simulink model "fft_biplex_real_4x_delay_bram_test"  (Simulink 7.4)
settings: Solver=VariableStepDiscrete  StartTime=0.0  StopTime=256  RelTol=1e-3
libraries: xbsIndex_r4 x596, casper_library_misc x36, casper_library_delays x8, casper_library_ffts_twiddle x1, simulink x1
(part 6 of 6)

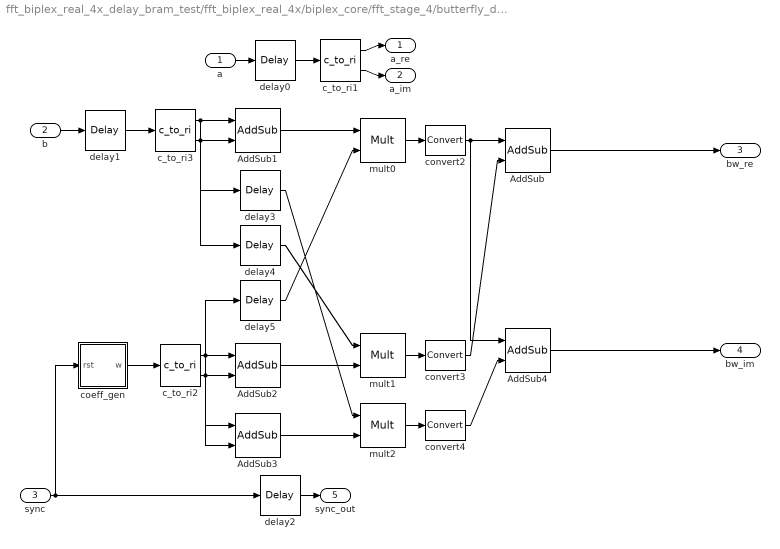
== system fft_biplex_real_4x_delay_bram_test/fft_biplex_real_4x/biplex_core/fft_stage_4/butterfly_direct/twiddle_general_3mult ==
  a : Inport
  b : Inport  Port=2
  sync : Inport  Port=3
  AddSub : xbsIndex_r4/AddSub  mode=Subtraction  use_carryin=off  use_carryout=off  en=off  latency=add_latency  precision=Full  arith_type=Unsigned  n_bits=16  bin_pt=14  quantization=Truncate  overflow=Wrap  dbl_ovrd=off  use_behavioral_HDL=on  hw_selection=Fabric  pipelined=off  block_type=addsub
  AddSub1 : xbsIndex_r4/AddSub  mode=Addition  use_carryin=off  use_carryout=off  en=off  latency=add_latency  precision=Full  arith_type=Unsigned  n_bits=16  bin_pt=14  quantization=Truncate  overflow=Wrap  dbl_ovrd=off  use_behavioral_HDL=on  hw_selection=Fabric  pipelined=off  block_type=addsub
  AddSub2 : xbsIndex_r4/AddSub  mode=Addition  use_carryin=off  use_carryout=off  en=off  latency=add_latency  precision=Full  arith_type=Unsigned  n_bits=16  bin_pt=14  quantization=Truncate  overflow=Wrap  dbl_ovrd=off  use_behavioral_HDL=on  hw_selection=Fabric  pipelined=off  block_type=addsub
  AddSub3 : xbsIndex_r4/AddSub  mode=Subtraction  use_carryin=off  use_carryout=off  en=off  latency=add_latency  precision=Full  arith_type=Unsigned  n_bits=16  bin_pt=14  quantization=Truncate  overflow=Wrap  dbl_ovrd=off  use_behavioral_HDL=on  hw_selection=Fabric  pipelined=off  block_type=addsub
  AddSub4 : xbsIndex_r4/AddSub  mode=Addition  use_carryin=off  use_carryout=off  en=off  latency=add_latency  precision=Full  arith_type=Unsigned  n_bits=16  bin_pt=14  quantization=Truncate  overflow=Wrap  dbl_ovrd=off  use_behavioral_HDL=on  hw_selection=Fabric  pipelined=off  block_type=addsub
  c_to_ri1 : casper_library_misc/c_to_ri  SystemSampleTime=-1  n_bits=16  bin_pt=15
      settings: AttributesFormatString=16_15 r/i
  c_to_ri2 : casper_library_misc/c_to_ri  SystemSampleTime=-1  n_bits=15  bin_pt=13
      settings: AttributesFormatString=15_13 r/i
  c_to_ri3 : casper_library_misc/c_to_ri  SystemSampleTime=-1  n_bits=input_bit_width  bin_pt=input_bit_width-1
      settings: AttributesFormatString=16_15 r/i
  coeff_gen : Subsystem  AncestorBlock=casper_library_ffts_twiddle_coeff_gen/coeff_gen  mask(coeff_gen){Coeffs=[1+0i                                        6.123233995736766035868820147292e-17-1i         0.70710678118654757273731092936941-0.70710678118654746171500846685376i        -0.70710678118654746171500846685376-0.70710678118654757273731092936941i         0.92387953251128673848313610506011-0.38268343236508978177923268049199i        -0.38268343236508972626808144923416-0.92387953251128673848313610506011i         0.38268343236508983729038391174981-0.92387953251128673848313610506011i        -0.92387953251128673848313610506011-0.38268343236508989280153514300764i], coeff_bit_width=15, StepPeriod=1, bram_latency=bram_latency, coeffs_bram=off}
      mask prompts: Coeffs "Coefficients: (0 to 2^(FFTSize-1)-1)"; coeff_bit_width "Coefficient Bit Width:"; StepPeriod "Step Period: (2^?)"; bram_latency "Latency:"; coeffs_bram "Store coefficients in BRAM"
      mask help: Generates a sequence of complex coefficients
      mask init:
      | coeff_gen_init( gcb, ...
      |     'Coeffs', Coeffs, ...
      |     'coeff_bit_width', coeff_bit_width, ...
      |     'StepPeriod', StepPeriod, ...
      |     'bram_latency', bram_latency, ...
      |     'coeffs_bram', coeffs_bram);
      settings: AttributesFormatString=8 @ (15,13)
      mask CallbackString:
      | Coeffs = eval(get_param(gcb, 'Coeffs'));
      | if( length(Coeffs) == 1 ),
      |     set_param(gcb, 'MaskVisibilities',{'on','on','off','off','off'});
      | else
      |     set_param(gcb, 'MaskVisibilities',{'on','on','on','on','on'});
      | end||||
  convert2 : xbsIndex_r4/Convert  arith_type="Signed  (2's comp)"  n_bits=input_bit_width+4  bin_pt=input_bit_width+1  quantization=Truncate  overflow=Saturate  latency=conv_latency  dbl_ovrd=off  pipeline=on  block_type=convert
      settings: block_version=11.4
  convert3 : xbsIndex_r4/Convert  arith_type="Signed  (2's comp)"  n_bits=input_bit_width+4  bin_pt=input_bit_width+1  quantization=Truncate  overflow=Saturate  latency=conv_latency  dbl_ovrd=off  pipeline=on  block_type=convert
      settings: block_version=11.4
  convert4 : xbsIndex_r4/Convert  arith_type="Signed  (2's comp)"  n_bits=input_bit_width+4  bin_pt=input_bit_width+1  quantization=Truncate  overflow=Saturate  latency=conv_latency  dbl_ovrd=off  pipeline=on  block_type=convert
      settings: block_version=11.4
  delay0 : xbsIndex_r4/Delay  en=off  latency=mult_latency + 2*add_latency + bram_latency + conv_latency  dbl_ovrd=off  reg_retiming=off  block_type=delay
      settings: block_version=11.4
  delay1 : xbsIndex_r4/Delay  en=off  latency=bram_latency  dbl_ovrd=off  reg_retiming=off  block_type=delay
      settings: block_version=11.4
  delay2 : xbsIndex_r4/Delay  en=off  latency=mult_latency + 2*add_latency + bram_latency + conv_latency  dbl_ovrd=off  reg_retiming=off  block_type=delay
      settings: block_version=11.4
  delay3 : xbsIndex_r4/Delay  en=off  latency=add_latency  dbl_ovrd=off  reg_retiming=on  block_type=delay
      settings: block_version=11.4
  delay4 : xbsIndex_r4/Delay  en=off  latency=add_latency  dbl_ovrd=off  reg_retiming=on  block_type=delay
      settings: block_version=11.4
  delay5 : xbsIndex_r4/Delay  en=off  latency=add_latency  dbl_ovrd=off  reg_retiming=on  block_type=delay
      settings: block_version=11.4
  mult0 : xbsIndex_r4/Mult  precision=Full  arith_type="Signed  (2's comp)"  n_bits=16  bin_pt=14  quantization=Truncate  overflow=Wrap  en=off  latency=mult_latency  dbl_ovrd=off  use_behavioral_HDL=on  opt=Speed  use_embedded=off  optimum_pipeline=off  pipeline=on  use_rpm=on  placement_style=Triangular  block_type=mult
      settings: block_version=11.4
  mult1 : xbsIndex_r4/Mult  precision=Full  arith_type="Signed  (2's comp)"  n_bits=16  bin_pt=14  quantization=Truncate  overflow=Wrap  en=off  latency=mult_latency  dbl_ovrd=off  use_behavioral_HDL=on  opt=Speed  use_embedded=off  optimum_pipeline=off  pipeline=on  use_rpm=on  placement_style=Triangular  block_type=mult
      settings: block_version=11.4
  mult2 : xbsIndex_r4/Mult  precision=Full  arith_type="Signed  (2's comp)"  n_bits=16  bin_pt=14  quantization=Truncate  overflow=Wrap  en=off  latency=mult_latency  dbl_ovrd=off  use_behavioral_HDL=on  opt=Speed  use_embedded=off  optimum_pipeline=off  pipeline=on  use_rpm=on  placement_style=Triangular  block_type=mult
      settings: block_version=11.4
  a_re : Outport
  a_im : Outport  Port=2
  bw_re : Outport  Port=3
  bw_im : Outport  Port=4
  sync_out : Outport  Port=5
  wires:
  a/1 -> delay0/1
  delay0/1 -> c_to_ri1/1
  c_to_ri1/1 -> a_re/1
  c_to_ri1/2 -> a_im/1
  sync/1 -> delay2/1, coeff_gen/1(rst)
  delay2/1 -> sync_out/1
  coeff_gen/1(w) -> c_to_ri2/1
  c_to_ri2/1 -> AddSub2/1, AddSub3/2, delay5/1
  c_to_ri2/2 -> AddSub2/2, AddSub3/1
  b/1 -> delay1/1
  delay1/1 -> c_to_ri3/1
  c_to_ri3/1 -> AddSub1/1, delay3/1
  c_to_ri3/2 -> AddSub1/2, delay4/1
  AddSub1/1 -> mult0/1
  delay5/1 -> mult0/2
  delay4/1 -> mult1/1
  AddSub2/1 -> mult1/2
  delay3/1 -> mult2/1
  AddSub3/1 -> mult2/2
  mult0/1 -> convert2/1
  mult1/1 -> convert3/1
  mult2/1 -> convert4/1
  convert2/1 -> AddSub/1, AddSub4/1
  convert3/1 -> AddSub/2
  convert4/1 -> AddSub4/2
  AddSub/1 -> bw_re/1
  AddSub4/1 -> bw_im/1

== system fft_biplex_real_4x_delay_bram_test/fft_biplex_real_4x/biplex_core/fft_stage_5/butterfly_direct/convert_of0 ==
  din : Inport  OutDataType=sfix(16)  OutScaling=2^0
  all_0s : xbsIndex_r4/Logical  logical_function=NAND  inputs=5  en=off  latency=latency  precision=Full  arith_type=Unsigned  n_bits=16  bin_pt=0  align_bp=on  dbl_ovrd=off  block_type=logical
  all_1s : xbsIndex_r4/Logical  logical_function=NAND  inputs=5  en=off  latency=latency  precision=Full  arith_type=Unsigned  n_bits=16  bin_pt=0  align_bp=on  dbl_ovrd=off  block_type=logical
  and : xbsIndex_r4/Logical  logical_function=AND  inputs=2  en=off  latency=0  precision=Full  arith_type=Unsigned  n_bits=16  bin_pt=0  align_bp=on  dbl_ovrd=off  block_type=logical
  convert : xbsIndex_r4/Convert  arith_type="Signed  (2's comp)"  n_bits=bit_width_o  bin_pt=binary_point_o  quantization=Truncate  overflow=Saturate  latency=latency  dbl_ovrd=off  pipeline=on  block_type=convert
      settings: block_version=10.1.1
  invert{1..5} (5 alike) : xbsIndex_r4/Inverter  en=off  latency=0  dbl_ovrd=off  block_type=inv
      invert3 settings: block_version=11.4
      invert4 settings: block_version=11.4
      invert5 settings: block_version=11.4
  slice1 : xbsIndex_r4/Slice  nbits=1  boolean_output=on  mode=Upper Bit Location + Width  bit1=0  base1=MSB of Input  bit0=0  base0=LSB of Input  dbl_ovrd=off  block_type=slice
      settings: infoedit="Extracts a given range of bits from each input sample and presents it at the output.  The output type is ordinarily unsigned with binary point at zero, but can be Boolean when the slice is one bit wide.<P><P>Hardware notes: In hardware this block costs nothing."  block_version=10.1.1
  slice2 : xbsIndex_r4/Slice  nbits=1  boolean_output=on  mode=Upper Bit Location + Width  bit1=-1  base1=MSB of Input  bit0=0  base0=LSB of Input  dbl_ovrd=off  block_type=slice
      settings: infoedit="Extracts a given range of bits from each input sample and presents it at the output.  The output type is ordinarily unsigned with binary point at zero, but can be Boolean when the slice is one bit wide.<P><P>Hardware notes: In hardware this block costs nothing."  block_version=10.1.1
  slice3 : xbsIndex_r4/Slice  nbits=1  boolean_output=on  mode=Upper Bit Location + Width  bit1=-2  base1=MSB of Input  bit0=0  base0=LSB of Input  dbl_ovrd=off  block_type=slice
  slice4 : xbsIndex_r4/Slice  nbits=1  boolean_output=on  mode=Upper Bit Location + Width  bit1=-3  base1=MSB of Input  bit0=0  base0=LSB of Input  dbl_ovrd=off  block_type=slice
  slice5 : xbsIndex_r4/Slice  nbits=1  boolean_output=on  mode=Upper Bit Location + Width  bit1=-4  base1=MSB of Input  bit0=0  base0=LSB of Input  dbl_ovrd=off  block_type=slice
  dout : Outport
  of : Outport  Port=2
  wires:
  din/1 -> convert/1, slice1/1, slice2/1, slice3/1, slice4/1, slice5/1
  convert/1 -> dout/1
  slice1/1 -> all_1s/1, invert1/1
  invert1/1 -> all_0s/1
  slice2/1 -> all_1s/2, invert2/1
  invert2/1 -> all_0s/2
  slice3/1 -> all_1s/3, invert3/1
  invert3/1 -> all_0s/3
  slice4/1 -> all_1s/4, invert4/1
  invert4/1 -> all_0s/4
  slice5/1 -> all_1s/5, invert5/1
  invert5/1 -> all_0s/5
  all_0s/1 -> and/1
  all_1s/1 -> and/2
  and/1 -> of/1

== system fft_biplex_real_4x_delay_bram_test/fft_biplex_real_4x/biplex_core/fft_stage_5/butterfly_direct/convert_of1 ==
  din : Inport  OutDataType=sfix(16)  OutScaling=2^0
  all_0s : xbsIndex_r4/Logical  logical_function=NAND  inputs=5  en=off  latency=latency  precision=Full  arith_type=Unsigned  n_bits=16  bin_pt=0  align_bp=on  dbl_ovrd=off  block_type=logical
  all_1s : xbsIndex_r4/Logical  logical_function=NAND  inputs=5  en=off  latency=latency  precision=Full  arith_type=Unsigned  n_bits=16  bin_pt=0  align_bp=on  dbl_ovrd=off  block_type=logical
  and : xbsIndex_r4/Logical  logical_function=AND  inputs=2  en=off  latency=0  precision=Full  arith_type=Unsigned  n_bits=16  bin_pt=0  align_bp=on  dbl_ovrd=off  block_type=logical
  convert : xbsIndex_r4/Convert  arith_type="Signed  (2's comp)"  n_bits=bit_width_o  bin_pt=binary_point_o  quantization=Truncate  overflow=Saturate  latency=latency  dbl_ovrd=off  pipeline=on  block_type=convert
      settings: block_version=10.1.1
  invert{1..5} (5 alike) : xbsIndex_r4/Inverter  en=off  latency=0  dbl_ovrd=off  block_type=inv
      invert3 settings: block_version=11.4
      invert4 settings: block_version=11.4
      invert5 settings: block_version=11.4
  slice1 : xbsIndex_r4/Slice  nbits=1  boolean_output=on  mode=Upper Bit Location + Width  bit1=0  base1=MSB of Input  bit0=0  base0=LSB of Input  dbl_ovrd=off  block_type=slice
      settings: infoedit="Extracts a given range of bits from each input sample and presents it at the output.  The output type is ordinarily unsigned with binary point at zero, but can be Boolean when the slice is one bit wide.<P><P>Hardware notes: In hardware this block costs nothing."  block_version=10.1.1
  slice2 : xbsIndex_r4/Slice  nbits=1  boolean_output=on  mode=Upper Bit Location + Width  bit1=-1  base1=MSB of Input  bit0=0  base0=LSB of Input  dbl_ovrd=off  block_type=slice
      settings: infoedit="Extracts a given range of bits from each input sample and presents it at the output.  The output type is ordinarily unsigned with binary point at zero, but can be Boolean when the slice is one bit wide.<P><P>Hardware notes: In hardware this block costs nothing."  block_version=10.1.1
  slice3 : xbsIndex_r4/Slice  nbits=1  boolean_output=on  mode=Upper Bit Location + Width  bit1=-2  base1=MSB of Input  bit0=0  base0=LSB of Input  dbl_ovrd=off  block_type=slice
  slice4 : xbsIndex_r4/Slice  nbits=1  boolean_output=on  mode=Upper Bit Location + Width  bit1=-3  base1=MSB of Input  bit0=0  base0=LSB of Input  dbl_ovrd=off  block_type=slice
  slice5 : xbsIndex_r4/Slice  nbits=1  boolean_output=on  mode=Upper Bit Location + Width  bit1=-4  base1=MSB of Input  bit0=0  base0=LSB of Input  dbl_ovrd=off  block_type=slice
  dout : Outport
  of : Outport  Port=2
  wires:
  din/1 -> convert/1, slice1/1, slice2/1, slice3/1, slice4/1, slice5/1
  convert/1 -> dout/1
  slice1/1 -> all_1s/1, invert1/1
  invert1/1 -> all_0s/1
  slice2/1 -> all_1s/2, invert2/1
  invert2/1 -> all_0s/2
  slice3/1 -> all_1s/3, invert3/1
  invert3/1 -> all_0s/3
  slice4/1 -> all_1s/4, invert4/1
  invert4/1 -> all_0s/4
  slice5/1 -> all_1s/5, invert5/1
  invert5/1 -> all_0s/5
  all_0s/1 -> and/1
  all_1s/1 -> and/2
  and/1 -> of/1

== system fft_biplex_real_4x_delay_bram_test/fft_biplex_real_4x/biplex_core/fft_stage_5/butterfly_direct/convert_of2 ==
  din : Inport  OutDataType=sfix(16)  OutScaling=2^0
  all_0s : xbsIndex_r4/Logical  logical_function=NAND  inputs=5  en=off  latency=latency  precision=Full  arith_type=Unsigned  n_bits=16  bin_pt=0  align_bp=on  dbl_ovrd=off  block_type=logical
  all_1s : xbsIndex_r4/Logical  logical_function=NAND  inputs=5  en=off  latency=latency  precision=Full  arith_type=Unsigned  n_bits=16  bin_pt=0  align_bp=on  dbl_ovrd=off  block_type=logical
  and : xbsIndex_r4/Logical  logical_function=AND  inputs=2  en=off  latency=0  precision=Full  arith_type=Unsigned  n_bits=16  bin_pt=0  align_bp=on  dbl_ovrd=off  block_type=logical
  convert : xbsIndex_r4/Convert  arith_type="Signed  (2's comp)"  n_bits=bit_width_o  bin_pt=binary_point_o  quantization=Truncate  overflow=Saturate  latency=latency  dbl_ovrd=off  pipeline=on  block_type=convert
      settings: block_version=10.1.1
  invert{1..5} (5 alike) : xbsIndex_r4/Inverter  en=off  latency=0  dbl_ovrd=off  block_type=inv
      invert3 settings: block_version=11.4
      invert4 settings: block_version=11.4
      invert5 settings: block_version=11.4
  slice1 : xbsIndex_r4/Slice  nbits=1  boolean_output=on  mode=Upper Bit Location + Width  bit1=0  base1=MSB of Input  bit0=0  base0=LSB of Input  dbl_ovrd=off  block_type=slice
      settings: infoedit="Extracts a given range of bits from each input sample and presents it at the output.  The output type is ordinarily unsigned with binary point at zero, but can be Boolean when the slice is one bit wide.<P><P>Hardware notes: In hardware this block costs nothing."  block_version=10.1.1
  slice2 : xbsIndex_r4/Slice  nbits=1  boolean_output=on  mode=Upper Bit Location + Width  bit1=-1  base1=MSB of Input  bit0=0  base0=LSB of Input  dbl_ovrd=off  block_type=slice
      settings: infoedit="Extracts a given range of bits from each input sample and presents it at the output.  The output type is ordinarily unsigned with binary point at zero, but can be Boolean when the slice is one bit wide.<P><P>Hardware notes: In hardware this block costs nothing."  block_version=10.1.1
  slice3 : xbsIndex_r4/Slice  nbits=1  boolean_output=on  mode=Upper Bit Location + Width  bit1=-2  base1=MSB of Input  bit0=0  base0=LSB of Input  dbl_ovrd=off  block_type=slice
  slice4 : xbsIndex_r4/Slice  nbits=1  boolean_output=on  mode=Upper Bit Location + Width  bit1=-3  base1=MSB of Input  bit0=0  base0=LSB of Input  dbl_ovrd=off  block_type=slice
  slice5 : xbsIndex_r4/Slice  nbits=1  boolean_output=on  mode=Upper Bit Location + Width  bit1=-4  base1=MSB of Input  bit0=0  base0=LSB of Input  dbl_ovrd=off  block_type=slice
  dout : Outport
  of : Outport  Port=2
  wires:
  din/1 -> convert/1, slice1/1, slice2/1, slice3/1, slice4/1, slice5/1
  convert/1 -> dout/1
  slice1/1 -> all_1s/1, invert1/1
  invert1/1 -> all_0s/1
  slice2/1 -> all_1s/2, invert2/1
  invert2/1 -> all_0s/2
  slice3/1 -> all_1s/3, invert3/1
  invert3/1 -> all_0s/3
  slice4/1 -> all_1s/4, invert4/1
  invert4/1 -> all_0s/4
  slice5/1 -> all_1s/5, invert5/1
  invert5/1 -> all_0s/5
  all_0s/1 -> and/1
  all_1s/1 -> and/2
  and/1 -> of/1

== system fft_biplex_real_4x_delay_bram_test/fft_biplex_real_4x/biplex_core/fft_stage_5/butterfly_direct/convert_of3 ==
  din : Inport  OutDataType=sfix(16)  OutScaling=2^0
  all_0s : xbsIndex_r4/Logical  logical_function=NAND  inputs=5  en=off  latency=latency  precision=Full  arith_type=Unsigned  n_bits=16  bin_pt=0  align_bp=on  dbl_ovrd=off  block_type=logical
  all_1s : xbsIndex_r4/Logical  logical_function=NAND  inputs=5  en=off  latency=latency  precision=Full  arith_type=Unsigned  n_bits=16  bin_pt=0  align_bp=on  dbl_ovrd=off  block_type=logical
  and : xbsIndex_r4/Logical  logical_function=AND  inputs=2  en=off  latency=0  precision=Full  arith_type=Unsigned  n_bits=16  bin_pt=0  align_bp=on  dbl_ovrd=off  block_type=logical
  convert : xbsIndex_r4/Convert  arith_type="Signed  (2's comp)"  n_bits=bit_width_o  bin_pt=binary_point_o  quantization=Truncate  overflow=Saturate  latency=latency  dbl_ovrd=off  pipeline=on  block_type=convert
      settings: block_version=10.1.1
  invert{1..5} (5 alike) : xbsIndex_r4/Inverter  en=off  latency=0  dbl_ovrd=off  block_type=inv
      invert3 settings: block_version=11.4
      invert4 settings: block_version=11.4
      invert5 settings: block_version=11.4
  slice1 : xbsIndex_r4/Slice  nbits=1  boolean_output=on  mode=Upper Bit Location + Width  bit1=0  base1=MSB of Input  bit0=0  base0=LSB of Input  dbl_ovrd=off  block_type=slice
      settings: infoedit="Extracts a given range of bits from each input sample and presents it at the output.  The output type is ordinarily unsigned with binary point at zero, but can be Boolean when the slice is one bit wide.<P><P>Hardware notes: In hardware this block costs nothing."  block_version=10.1.1
  slice2 : xbsIndex_r4/Slice  nbits=1  boolean_output=on  mode=Upper Bit Location + Width  bit1=-1  base1=MSB of Input  bit0=0  base0=LSB of Input  dbl_ovrd=off  block_type=slice
      settings: infoedit="Extracts a given range of bits from each input sample and presents it at the output.  The output type is ordinarily unsigned with binary point at zero, but can be Boolean when the slice is one bit wide.<P><P>Hardware notes: In hardware this block costs nothing."  block_version=10.1.1
  slice3 : xbsIndex_r4/Slice  nbits=1  boolean_output=on  mode=Upper Bit Location + Width  bit1=-2  base1=MSB of Input  bit0=0  base0=LSB of Input  dbl_ovrd=off  block_type=slice
  slice4 : xbsIndex_r4/Slice  nbits=1  boolean_output=on  mode=Upper Bit Location + Width  bit1=-3  base1=MSB of Input  bit0=0  base0=LSB of Input  dbl_ovrd=off  block_type=slice
  slice5 : xbsIndex_r4/Slice  nbits=1  boolean_output=on  mode=Upper Bit Location + Width  bit1=-4  base1=MSB of Input  bit0=0  base0=LSB of Input  dbl_ovrd=off  block_type=slice
  dout : Outport
  of : Outport  Port=2
  wires:
  din/1 -> convert/1, slice1/1, slice2/1, slice3/1, slice4/1, slice5/1
  convert/1 -> dout/1
  slice1/1 -> all_1s/1, invert1/1
  invert1/1 -> all_0s/1
  slice2/1 -> all_1s/2, invert2/1
  invert2/1 -> all_0s/2
  slice3/1 -> all_1s/3, invert3/1
  invert3/1 -> all_0s/3
  slice4/1 -> all_1s/4, invert4/1
  invert4/1 -> all_0s/4
  slice5/1 -> all_1s/5, invert5/1
  invert5/1 -> all_0s/5
  all_0s/1 -> and/1
  all_1s/1 -> and/2
  and/1 -> of/1

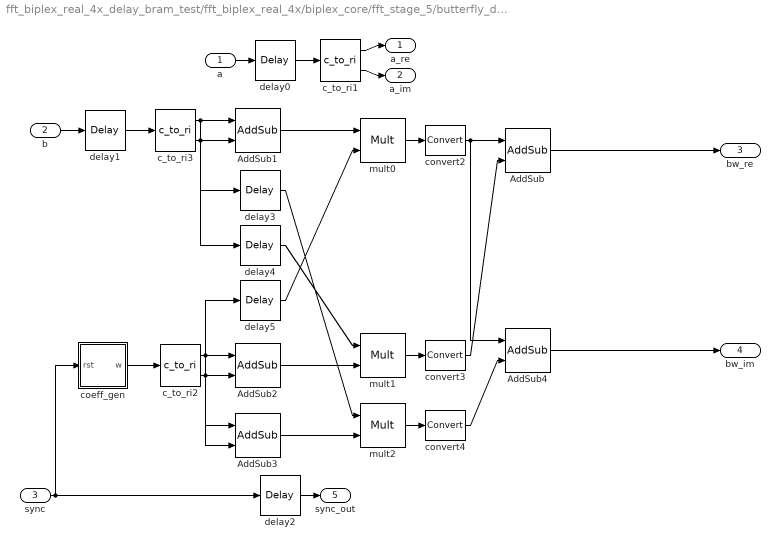
== system fft_biplex_real_4x_delay_bram_test/fft_biplex_real_4x/biplex_core/fft_stage_5/butterfly_direct/twiddle_general_3mult ==
  a : Inport
  b : Inport  Port=2
  sync : Inport  Port=3
  AddSub : xbsIndex_r4/AddSub  mode=Subtraction  use_carryin=off  use_carryout=off  en=off  latency=add_latency  precision=Full  arith_type=Unsigned  n_bits=16  bin_pt=14  quantization=Truncate  overflow=Wrap  dbl_ovrd=off  use_behavioral_HDL=on  hw_selection=Fabric  pipelined=off  block_type=addsub
  AddSub1 : xbsIndex_r4/AddSub  mode=Addition  use_carryin=off  use_carryout=off  en=off  latency=add_latency  precision=Full  arith_type=Unsigned  n_bits=16  bin_pt=14  quantization=Truncate  overflow=Wrap  dbl_ovrd=off  use_behavioral_HDL=on  hw_selection=Fabric  pipelined=off  block_type=addsub
  AddSub2 : xbsIndex_r4/AddSub  mode=Addition  use_carryin=off  use_carryout=off  en=off  latency=add_latency  precision=Full  arith_type=Unsigned  n_bits=16  bin_pt=14  quantization=Truncate  overflow=Wrap  dbl_ovrd=off  use_behavioral_HDL=on  hw_selection=Fabric  pipelined=off  block_type=addsub
  AddSub3 : xbsIndex_r4/AddSub  mode=Subtraction  use_carryin=off  use_carryout=off  en=off  latency=add_latency  precision=Full  arith_type=Unsigned  n_bits=16  bin_pt=14  quantization=Truncate  overflow=Wrap  dbl_ovrd=off  use_behavioral_HDL=on  hw_selection=Fabric  pipelined=off  block_type=addsub
  AddSub4 : xbsIndex_r4/AddSub  mode=Addition  use_carryin=off  use_carryout=off  en=off  latency=add_latency  precision=Full  arith_type=Unsigned  n_bits=16  bin_pt=14  quantization=Truncate  overflow=Wrap  dbl_ovrd=off  use_behavioral_HDL=on  hw_selection=Fabric  pipelined=off  block_type=addsub
  c_to_ri1 : casper_library_misc/c_to_ri  SystemSampleTime=-1  n_bits=16  bin_pt=15
      settings: AttributesFormatString=16_15 r/i
  c_to_ri2 : casper_library_misc/c_to_ri  SystemSampleTime=-1  n_bits=15  bin_pt=13
      settings: AttributesFormatString=15_13 r/i
  c_to_ri3 : casper_library_misc/c_to_ri  SystemSampleTime=-1  n_bits=input_bit_width  bin_pt=input_bit_width-1
      settings: AttributesFormatString=16_15 r/i
  coeff_gen : Subsystem  AncestorBlock=casper_library_ffts_twiddle_coeff_gen/coeff_gen  mask(coeff_gen){Coeffs=[1+0i                                        6.123233995736766035868820147292e-17-1i         0.70710678118654757273731092936941-0.70710678118654746171500846685376i        -0.70710678118654746171500846685376-0.70710678118654757273731092936941i         0.92387953251128673848313610506011-0.38268343236508978177923268049199i        -0.38268343236508972626808144923416-0.92387953251128673848313610506011i         0.38268343236508983729038391174981-0.92387953251128673848313610506011i        -0.92387953251128673848313610506011-0.38268343236508989280153514300764i         0.98078528040323043057924223830923-0.19509032201612824808378832130984i        -0.19509032201612819257263709005201-0.98078528040323043057924223830923i          0.55557023301960228867102387084742-0.8314696123025452356714026791451i        -0.83146961230254534669370514166076-0.55557023301960217764872140833177i          0.8314696123025452356714026791451-0.55557023301960217764872140833177i        -0.55557023301960195560411648330046-0.83146961230254534669370514166076i         0.19509032201612833135051516819658-0.98078528040323043057924223830923i        -0.98078528040323043057924223830923-0.19509032201612860890627132448572i], coeff_bit_width=15, StepPeriod=0, bram_latency=bram_latency, coeffs_bram=off}
      mask prompts: Coeffs "Coefficients: (0 to 2^(FFTSize-1)-1)"; coeff_bit_width "Coefficient Bit Width:"; StepPeriod "Step Period: (2^?)"; bram_latency "Latency:"; coeffs_bram "Store coefficients in BRAM"
      mask help: Generates a sequence of complex coefficients
      mask init:
      | coeff_gen_init( gcb, ...
      |     'Coeffs', Coeffs, ...
      |     'coeff_bit_width', coeff_bit_width, ...
      |     'StepPeriod', StepPeriod, ...
      |     'bram_latency', bram_latency, ...
      |     'coeffs_bram', coeffs_bram);
      settings: AttributesFormatString=16 @ (15,13)
      mask CallbackString:
      | Coeffs = eval(get_param(gcb, 'Coeffs'));
      | if( length(Coeffs) == 1 ),
      |     set_param(gcb, 'MaskVisibilities',{'on','on','off','off','off'});
      | else
      |     set_param(gcb, 'MaskVisibilities',{'on','on','on','on','on'});
      | end||||
  convert2 : xbsIndex_r4/Convert  arith_type="Signed  (2's comp)"  n_bits=input_bit_width+4  bin_pt=input_bit_width+1  quantization=Truncate  overflow=Saturate  latency=conv_latency  dbl_ovrd=off  pipeline=on  block_type=convert
      settings: block_version=11.4
  convert3 : xbsIndex_r4/Convert  arith_type="Signed  (2's comp)"  n_bits=input_bit_width+4  bin_pt=input_bit_width+1  quantization=Truncate  overflow=Saturate  latency=conv_latency  dbl_ovrd=off  pipeline=on  block_type=convert
      settings: block_version=11.4
  convert4 : xbsIndex_r4/Convert  arith_type="Signed  (2's comp)"  n_bits=input_bit_width+4  bin_pt=input_bit_width+1  quantization=Truncate  overflow=Saturate  latency=conv_latency  dbl_ovrd=off  pipeline=on  block_type=convert
      settings: block_version=11.4
  delay0 : xbsIndex_r4/Delay  en=off  latency=mult_latency + 2*add_latency + bram_latency + conv_latency  dbl_ovrd=off  reg_retiming=off  block_type=delay
      settings: block_version=11.4
  delay1 : xbsIndex_r4/Delay  en=off  latency=bram_latency  dbl_ovrd=off  reg_retiming=off  block_type=delay
      settings: block_version=11.4
  delay2 : xbsIndex_r4/Delay  en=off  latency=mult_latency + 2*add_latency + bram_latency + conv_latency  dbl_ovrd=off  reg_retiming=off  block_type=delay
      settings: block_version=11.4
  delay3 : xbsIndex_r4/Delay  en=off  latency=add_latency  dbl_ovrd=off  reg_retiming=on  block_type=delay
      settings: block_version=11.4
  delay4 : xbsIndex_r4/Delay  en=off  latency=add_latency  dbl_ovrd=off  reg_retiming=on  block_type=delay
      settings: block_version=11.4
  delay5 : xbsIndex_r4/Delay  en=off  latency=add_latency  dbl_ovrd=off  reg_retiming=on  block_type=delay
      settings: block_version=11.4
  mult0 : xbsIndex_r4/Mult  precision=Full  arith_type="Signed  (2's comp)"  n_bits=16  bin_pt=14  quantization=Truncate  overflow=Wrap  en=off  latency=mult_latency  dbl_ovrd=off  use_behavioral_HDL=off  opt=Speed  use_embedded=on  optimum_pipeline=off  pipeline=on  use_rpm=on  placement_style=Triangular  block_type=mult
      settings: block_version=11.4
  mult1 : xbsIndex_r4/Mult  precision=Full  arith_type="Signed  (2's comp)"  n_bits=16  bin_pt=14  quantization=Truncate  overflow=Wrap  en=off  latency=mult_latency  dbl_ovrd=off  use_behavioral_HDL=off  opt=Speed  use_embedded=on  optimum_pipeline=off  pipeline=on  use_rpm=on  placement_style=Triangular  block_type=mult
      settings: block_version=11.4
  mult2 : xbsIndex_r4/Mult  precision=Full  arith_type="Signed  (2's comp)"  n_bits=16  bin_pt=14  quantization=Truncate  overflow=Wrap  en=off  latency=mult_latency  dbl_ovrd=off  use_behavioral_HDL=off  opt=Speed  use_embedded=on  optimum_pipeline=off  pipeline=on  use_rpm=on  placement_style=Triangular  block_type=mult
      settings: block_version=11.4
  a_re : Outport
  a_im : Outport  Port=2
  bw_re : Outport  Port=3
  bw_im : Outport  Port=4
  sync_out : Outport  Port=5
  wires:
  a/1 -> delay0/1
  delay0/1 -> c_to_ri1/1
  c_to_ri1/1 -> a_re/1
  c_to_ri1/2 -> a_im/1
  sync/1 -> delay2/1, coeff_gen/1(rst)
  delay2/1 -> sync_out/1
  coeff_gen/1(w) -> c_to_ri2/1
  c_to_ri2/1 -> AddSub2/1, AddSub3/2, delay5/1
  c_to_ri2/2 -> AddSub2/2, AddSub3/1
  b/1 -> delay1/1
  delay1/1 -> c_to_ri3/1
  c_to_ri3/1 -> AddSub1/1, delay3/1
  c_to_ri3/2 -> AddSub1/2, delay4/1
  AddSub1/1 -> mult0/1
  delay5/1 -> mult0/2
  delay4/1 -> mult1/1
  AddSub2/1 -> mult1/2
  delay3/1 -> mult2/1
  AddSub3/1 -> mult2/2
  mult0/1 -> convert2/1
  mult1/1 -> convert3/1
  mult2/1 -> convert4/1
  convert2/1 -> AddSub/1, AddSub4/1
  convert3/1 -> AddSub/2
  convert4/1 -> AddSub4/2
  AddSub/1 -> bw_re/1
  AddSub4/1 -> bw_im/1

== system fft_biplex_real_4x_delay_bram_test/fft_biplex_real_4x/biplex_core/fft_stage_3/butterfly_direct/twiddle_general_3mult/coeff_gen ==
  rst : Inport
  Counter : xbsIndex_r4/Counter  cnt_type=Free Running  cnt_to=Inf  operation=Up  start_count=0  cnt_by_val=1  arith_type=Unsigned  n_bits=4  bin_pt=0  load_pin=off  rst=on  en=off  explicit_period=on  period=1  dbl_ovrd=off  use_behavioral_HDL=off  implementation=Fabric  block_type=counter
      settings: block_version=11.4
  ROM : xbsIndex_r4/ROM  depth=4  initVector="[1                                      0                        0.7071533203125                       -0.7071533203125]"  distributed_mem=Distributed memory  rst=off  init_reg=0  en=off  latency=1  arith_type="Signed  (2's comp)"  n_bits=15  bin_pt=13  dbl_ovrd=off  optimize=Area  use_rpm=on  block_type=sprom
      settings: block_version=11.4
  ROM1 : xbsIndex_r4/ROM  depth=4  initVector="[0                                     -1                       -0.7071533203125                       -0.7071533203125]"  distributed_mem=Distributed memory  rst=off  init_reg=0  en=off  latency=1  arith_type="Signed  (2's comp)"  n_bits=15  bin_pt=13  dbl_ovrd=off  optimize=Area  use_rpm=on  block_type=sprom
      settings: block_version=11.4
  Slice : xbsIndex_r4/Slice  nbits=2  boolean_output=off  mode=Upper Bit Location + Width  bit1=0  base1=MSB of Input  bit0=0  base0=LSB of Input  dbl_ovrd=off  block_type=slice
  ri_to_c : casper_library_misc/ri_to_c  SystemSampleTime=-1
  w : Outport
  wires:
  ri_to_c/1 -> w/1
  rst/1 -> Counter/1
  Counter/1 -> Slice/1
  Slice/1 -> ROM/1, ROM1/1
  ROM/1 -> ri_to_c/1
  ROM1/1 -> ri_to_c/2

== system fft_biplex_real_4x_delay_bram_test/fft_biplex_real_4x/biplex_core/fft_stage_4/butterfly_direct/twiddle_general_3mult/coeff_gen ==
  rst : Inport
  Counter : xbsIndex_r4/Counter  cnt_type=Free Running  cnt_to=Inf  operation=Up  start_count=0  cnt_by_val=1  arith_type=Unsigned  n_bits=4  bin_pt=0  load_pin=off  rst=on  en=off  explicit_period=on  period=1  dbl_ovrd=off  use_behavioral_HDL=off  implementation=Fabric  block_type=counter
      settings: block_version=11.4
  ROM : xbsIndex_r4/ROM  depth=8  initVector="[1                                      0                        0.7071533203125                       -0.7071533203125                            0.923828125                       -0.3826904296875                        0.3826904296875                           -0.923828125]"  distributed_mem=Distributed memory  rst=off  init_reg=0  en=off  latency=1  arith_type="Signed  (2's comp)"  n_bits=15  bin_pt=13  dbl_ovrd=off  optimize=Area  use_rpm=on  block_type=sprom
      settings: block_version=11.4
  ROM1 : xbsIndex_r4/ROM  depth=8  initVector="[0                                     -1                       -0.7071533203125                       -0.7071533203125                       -0.3826904296875                           -0.923828125                           -0.923828125                       -0.3826904296875]"  distributed_mem=Distributed memory  rst=off  init_reg=0  en=off  latency=1  arith_type="Signed  (2's comp)"  n_bits=15  bin_pt=13  dbl_ovrd=off  optimize=Area  use_rpm=on  block_type=sprom
      settings: block_version=11.4
  Slice : xbsIndex_r4/Slice  nbits=3  boolean_output=off  mode=Upper Bit Location + Width  bit1=0  base1=MSB of Input  bit0=0  base0=LSB of Input  dbl_ovrd=off  block_type=slice
  ri_to_c : casper_library_misc/ri_to_c  SystemSampleTime=-1
  w : Outport
  wires:
  ri_to_c/1 -> w/1
  rst/1 -> Counter/1
  Counter/1 -> Slice/1
  Slice/1 -> ROM/1, ROM1/1
  ROM/1 -> ri_to_c/1
  ROM1/1 -> ri_to_c/2

== system fft_biplex_real_4x_delay_bram_test/fft_biplex_real_4x/biplex_core/fft_stage_5/butterfly_direct/twiddle_general_3mult/coeff_gen ==
  rst : Inport
  Counter : xbsIndex_r4/Counter  cnt_type=Free Running  cnt_to=Inf  operation=Up  start_count=0  cnt_by_val=1  arith_type=Unsigned  n_bits=4  bin_pt=0  load_pin=off  rst=on  en=off  explicit_period=on  period=1  dbl_ovrd=off  use_behavioral_HDL=off  implementation=Fabric  block_type=counter
      settings: block_version=11.4
  ROM : xbsIndex_r4/ROM  depth=16  initVector="[1                                      0                        0.7071533203125                       -0.7071533203125                            0.923828125                       -0.3826904296875                        0.3826904296875                           -0.923828125                        0.9808349609375                        -0.195068359375                        0.5555419921875                       -0.8314208984375                        0.8314208984375                       -0.5555419921875                         0.195068359375                       -0.9808349609375]"  distributed_mem=Distributed memory  rst=off  init_reg=0  en=off  latency=1  arith_type="Signed  (2's comp)"  n_bits=15  bin_pt=13  dbl_ovrd=off  optimize=Area  use_rpm=on  block_type=sprom
      settings: block_version=11.4
  ROM1 : xbsIndex_r4/ROM  depth=16  initVector="[0                                     -1                       -0.7071533203125                       -0.7071533203125                       -0.3826904296875                           -0.923828125                           -0.923828125                       -0.3826904296875                        -0.195068359375                       -0.9808349609375                       -0.8314208984375                       -0.5555419921875                       -0.5555419921875                       -0.8314208984375                       -0.9808349609375                        -0.195068359375]"  distributed_mem=Distributed memory  rst=off  init_reg=0  en=off  latency=1  arith_type="Signed  (2's comp)"  n_bits=15  bin_pt=13  dbl_ovrd=off  optimize=Area  use_rpm=on  block_type=sprom
      settings: block_version=11.4
  Slice : xbsIndex_r4/Slice  nbits=4  boolean_output=off  mode=Upper Bit Location + Width  bit1=0  base1=MSB of Input  bit0=0  base0=LSB of Input  dbl_ovrd=off  block_type=slice
  ri_to_c : casper_library_misc/ri_to_c  SystemSampleTime=-1
  w : Outport
  wires:
  ri_to_c/1 -> w/1
  rst/1 -> Counter/1
  Counter/1 -> Slice/1
  Slice/1 -> ROM/1, ROM1/1
  ROM/1 -> ri_to_c/1
  ROM1/1 -> ri_to_c/2
